simulink model "asm_blocks_lib"  (R2026b)
settings: Solver=VariableStepAuto
libraries: nesl_utility x45, asmlib_lib x25, fl_lib x3, ee_lib x3
(part 1 of 3)
settings Model: Creator=fsbb  LastModifiedBy=fsbb

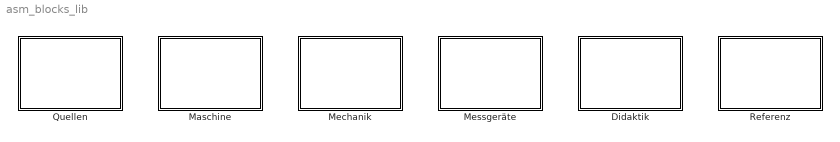
== system asm_blocks_lib ==
  Didaktik : Subsystem
      mask Display: disp('Didaktik');
  Maschine : Subsystem
      mask Display: disp('Maschine');
  Mechanik : Subsystem
      mask Display: disp('Mechanik');
  Messgeräte : Subsystem
      mask Display: disp('Messgeräte');
  Quellen : Subsystem
      mask Display: disp('Quellen');
  Referenz : Subsystem
      mask Display: disp('Referenz');

== system asm_blocks_lib/Didaktik ==
  Drehfeld-Anzeige : Subsystem  Tag=asmlib:field_display  mask(ASM-Bibliothek: Drehfeld-Anzeige){view_frame=rotorfest, image_orientation=wie Folien (U1 oben, Feld im Uhrzeigersinn), decomposition=on, change_vector=on, force_arrows=on, all_bars=on, slow_motion=0.05, N2=28, p=2, l=0.15, r=0.06, N1xi1=144, bar1_angle=-90}
      mask prompts: view_frame "Ansicht"; image_orientation "Orientierung"; decomposition "Feldzerlegung B⊥ / B∥ zeigen (Folie 16)"; change_vector "Änderungsvektor zeigen (Folie 17)"; force_arrows "Kraftpfeile zeigen (Folie 19)"; all_bars "alle Stäbe zeigen"; slow_motion "Zeitlupe (Simulationszeit je Sekunde Abspielzeit) [s]"; N2 "Anzahl Rotorstäbe N2 (2 = nur die Leiterschleife) [-]"; p "Polpaarzahl p [-]"; l "wirksame Stablänge l [m]"; r "Radius der Stabmitte r [m]"; N1xi1 "wirksame Windungszahl N1·ξ1 [-]"; bar1_angle "mechanische Lage von Stab 1 (0 = Achse Strang U, −90 = in der Folienansicht oben) [°]"
      mask help:
      | Rotorquerschnitt mit Drehfeld, Stabströmen und Kräften im Stil der Folien 16-30. Der Baustein
      | protokolliert ψh, i2′, ϑ in out.field_display_log (ein Baustein je Modell); nach der Simulation
      | startet der Knopf "Animation zeigen" die Animation (asmtools.field_animation). Einzelbilder
      | für Folien: asmexport.cross_section_series. Feldzerlegung und Änderungsvektor nur bei p = 1.
      |
      | Gleichungen:
      |   φ_el = ∠ψh,   B̂ = p·|ψh| / (2·N1ξ1·l·r),   B(γ,t) = B̂·cos(γ − φ_el)
      |   γ_k = p·ϑ + (k−1)·2π·p/N2,   î_Stab = 6·N1ξ1/N2·|i2′|,   ε2 = ∠i2′
      |   i_k = î_Stab·sin(γ_k − ε2) = î_Stab·sin(γ_k − φ_el + φ2),   φ2 = ∠ψh − ∠i2′
      |   B_k = B̂·cos(γ_k − φ_el),   F_k = i_k·l·B_k,   M_k = F_k·r
      |   Darstellung wie Folien: i_k,Folie = −i_k (positiv aus der Zeichenebene)
      |
      | Quelle: Hagl, R.: Elektrische Antriebstechnik. Hanser, München 2013; Densborn, Skript "DS-Asynchron-Motor" (DHBW Mannheim), Folien 16-30
      mask Help:
      | Rotorquerschnitt mit Drehfeld, Stabströmen und Kräften im Stil der Folien 16-30. Der Baustein
      | protokolliert ψh, i2′, ϑ in out.field_display_log (ein Baustein je Modell); nach der Simulation
      | startet der Knopf "Animation zeigen" die Animation (asmtools.field_animation). Einzelbilder
      | für Folien: asmexport.cross_section_series. Feldzerlegung und Änderungsvektor nur bei p = 1.
      | 
      | Gleichungen:
      |   φ_el = ∠ψh,   B̂ = p·|ψh| / (2·N1ξ1·l·r),   B(γ,t) = B̂·cos(γ − φ_el)
      |   γ_k = p·ϑ + (k−1)·2π·p/N2,   î_Stab = 6·N1ξ1/N2·|i2′|,   ε2 = ∠i2′
      |   i_k = î_Stab·sin(γ_k − ε2) = î_Stab·sin(γ_k − φ_el + φ2),   φ2 = ∠ψh − ∠i2′
      |   B_k = B̂·cos(γ_k − φ_el),   F_k = i_k·l·B_k,   M_k = F_k·r
      |   Darstellung wie Folien: i_k,Folie = −i_k (positiv aus der Zeichenebene)
      | 
      | Quelle: Hagl, R.: Elektrische Antriebstechnik. Hanser, München 2013; Densborn, Skript "DS-Asynchron-Motor" (DHBW Mannheim), Folien 16-30
      | 
      | Parameter und Wertebereiche:
      |   view_frame     Auswahl: rotorfest | statorfest
      |   image_orientation Auswahl: wie Folien (U1 oben, Feld im Uhrzeigersinn) | mathematisch positiv
      |   decomposition  ein/aus
      |   change_vector  ein/aus
      |   force_arrows   ein/aus
      |   all_bars       ein/aus
      |   slow_motion    > 0  [s]
      |   N2             ganzzahlig, ≥ 2  [-]
      |   p              ganzzahlig, ≥ 1, ≤ 12  [-]
      |   l              > 0  [m]
      |   r              > 0  [m]
      |   N1xi1          > 0  [-]
      |   bar1_angle     ≥ -360, ≤ 360  [°]
      | 
      | Alle Standardwerte sind Beispielwerte (parameter/asm_standard.m), keine Datenblattwerte.
      | Spezifikation: doku/SPEC.md
      mask TypeOptions view_frame: rotorfest | statorfest
      mask TypeOptions image_orientation: wie Folien (U1 oben, Feld im Uhrzeigersinn) | mathematisch positiv
      mask DialogControl evaluation_button Prompt: Animation zeigen
      mask DialogControl evaluation_button Callback: asmtools.field_animation(gcb);
      mask Display:
      | plot([0.1 0.9 0.9 0.1 0.1], [0.15 0.15 0.85 0.85 0.15]);
      | text(0.5, 0.5, 'Anzeige', 'horizontalAlignment', 'center', 'verticalAlignment', 'middle', 'texmode', 'on');
      | port_label('input', 1, '\psi_h', 'texmode', 'on');
      | port_label('input', 2, 'i2b', 'texmode', 'on');
      | port_label('input', 3, '\vartheta_{mech}', 'texmode', 'on');
  Ideales Drehfeld : Subsystem  Tag=asmlib:ideal_field  mask(ASM-Bibliothek: Ideales Drehfeld){Bhat=0.8, f1=50, p=2, s=1, l=0.15, r=0.06, N1xi1=144, N2=28, R2_S=0.000318664, L2s_S=5.0717e-06, phi2_mode=aus Rotorimpedanz (φ2 = 90° + φZ), phi2_fix=90}
      mask prompts: Bhat "Amplitude der Luftspaltflussdichte B̂ [T]"; f1 "Statorfrequenz f1 [Hz]"; p "Polpaarzahl p [-]"; s "Schlupf s [-]"; l "wirksame Stablänge l [m]"; r "Radius der Stabmitte r [m]"; N1xi1 "wirksame Windungszahl N1·ξ1 [-]"; N2 "Anzahl Rotorstäbe N2 (2 = nur die Leiterschleife) [-]"; R2_S "Widerstand einer Leiterschleife R2 [Ω]"; L2s_S "Streuinduktivität einer Leiterschleife L2σ [H]"; phi2_mode "Versatzwinkel φ2"; phi2_fix "fester Versatzwinkel φ2 [°]"
      mask help:
      | Kinematische Quelle wie Teil A des Prototyps: Drehfeld mit konstanter Amplitude, Rotor mit festem Schlupf.
      | Liefert dieselben Signale wie der Motor (ψh, i2′, ϑ), damit Rotorstab-Sonde und Drehfeld-Anzeige
      | ohne Motor betrieben werden können (Folien 16-30: s = 1, φ2 = 90°).
      |
      | Gleichungen:
      |   θ2 = ∫ s·ω1 dt,  U20 = 2·B̂·l·ω1·r/p,  î2 = s·U20/√(R2² + (s·ω1·L2σ)²)
      |   φZ = arctan(s·ω1·L2σ/R2),  φ2 = 90° + φZ  oder  φ2 = φ2,fix
      |
      | Quelle: Hagl, R.: Elektrische Antriebstechnik. Hanser, München 2013; Densborn, Skript "DS-Asynchron-Motor" (DHBW Mannheim), Folien 14-30
      mask Help:
      | Kinematische Quelle wie Teil A des Prototyps: Drehfeld mit konstanter Amplitude, Rotor mit festem Schlupf.
      | Liefert dieselben Signale wie der Motor (ψh, i2′, ϑ), damit Rotorstab-Sonde und Drehfeld-Anzeige
      | ohne Motor betrieben werden können (Folien 16-30: s = 1, φ2 = 90°).
      | 
      | Gleichungen:
      |   θ2 = ∫ s·ω1 dt,  U20 = 2·B̂·l·ω1·r/p,  î2 = s·U20/√(R2² + (s·ω1·L2σ)²)
      |   φZ = arctan(s·ω1·L2σ/R2),  φ2 = 90° + φZ  oder  φ2 = φ2,fix
      | 
      | Quelle: Hagl, R.: Elektrische Antriebstechnik. Hanser, München 2013; Densborn, Skript "DS-Asynchron-Motor" (DHBW Mannheim), Folien 14-30
      | 
      | Parameter und Wertebereiche:
      |   Bhat           > 0, ≤ 2.5  [T]
      |   f1             > 0, ≤ 1000  [Hz]
      |   p              ganzzahlig, ≥ 1, ≤ 12  [-]
      |   s              ≥ -1, ≤ 2  [-]
      |   l              > 0  [m]
      |   r              > 0  [m]
      |   N1xi1          > 0  [-]
      |   N2             ganzzahlig, ≥ 2  [-]
      |   R2_S           > 0  [Ω]
      |   L2s_S          > 0  [H]
      |   phi2_mode      Auswahl: aus Rotorimpedanz (φ2 = 90° + φZ) | fest
      |   phi2_fix       ≥ 0, ≤ 180  [°]
      | 
      | Alle Standardwerte sind Beispielwerte (parameter/asm_standard.m), keine Datenblattwerte.
      | Spezifikation: doku/SPEC.md
      mask TypeOptions phi2_mode: aus Rotorimpedanz (φ2 = 90° + φZ) | fest
      mask Display:
      | plot([0.1 0.9 0.9 0.1 0.1], [0.15 0.15 0.85 0.85 0.15]);
      | text(0.5, 0.5, 'Drehfeld', 'horizontalAlignment', 'center', 'verticalAlignment', 'middle', 'texmode', 'on');
      | port_label('output', 1, '\psi_h', 'texmode', 'on');
      | port_label('output', 2, 'i2b', 'texmode', 'on');
      | port_label('output', 3, '\vartheta_{mech}', 'texmode', 'on');
      | port_label('output', 4, '\phi_{el}', 'texmode', 'on');
      | port_label('output', 5, '\phi2', 'texmode', 'on');
  Kennlinienschreiber : Subsystem  Tag=asmlib:torque_speed_recorder  mask(ASM-Bibliothek: Kennlinienschreiber){show_kloss=on, show_ec=off, MK=71.55, sK=0.2, ns=1500}
      mask prompts: show_kloss "Kloss-Kennlinie einzeichnen"; show_ec "stationäre ESB-Kennlinie einzeichnen"; MK "Kippmoment MK [N·m]"; sK "Kippschlupf sK [-]"; ns "Synchrondrehzahl ns [1/min]"
      mask help:
      | Protokolliert n, M und M_L in out.torque_speed_log (ein Baustein je Modell). Der Knopf "Kennlinie
      | zeichnen" zeigt nach der Simulation das M(n)-Diagramm mit stationären Kennlinien und
      | Arbeitspunkt (asmtools.torque_speed_plot).
      |
      | Gleichungen:
      |   M = 2·MK·s·sK / (s² + sK²),   s = (ns − n)/ns
      |
      | Quelle: Hagl, R.: Elektrische Antriebstechnik. Hanser, München 2013; Densborn, Skript "DS-Asynchron-Motor" (DHBW Mannheim), Folien 47-56
      mask Help:
      | Protokolliert n, M und M_L in out.torque_speed_log (ein Baustein je Modell). Der Knopf "Kennlinie
      | zeichnen" zeigt nach der Simulation das M(n)-Diagramm mit stationären Kennlinien und
      | Arbeitspunkt (asmtools.torque_speed_plot).
      | 
      | Gleichungen:
      |   M = 2·MK·s·sK / (s² + sK²),   s = (ns − n)/ns
      | 
      | Quelle: Hagl, R.: Elektrische Antriebstechnik. Hanser, München 2013; Densborn, Skript "DS-Asynchron-Motor" (DHBW Mannheim), Folien 47-56
      | 
      | Parameter und Wertebereiche:
      |   show_kloss     ein/aus
      |   show_ec        ein/aus
      |   MK             > 0  [N·m]
      |   sK             > 0, ≤ 1  [-]
      |   ns             > 0  [1/min]
      | 
      | Alle Standardwerte sind Beispielwerte (parameter/asm_standard.m), keine Datenblattwerte.
      | Spezifikation: doku/SPEC.md
      mask DialogControl evaluation_button Prompt: Kennlinie zeichnen
      mask DialogControl evaluation_button Callback: asmtools.torque_speed_plot(gcb);
      mask Display:
      | plot([0.1 0.9 0.9 0.1 0.1], [0.15 0.15 0.85 0.85 0.15]);
      | text(0.5, 0.5, 'M(n)', 'horizontalAlignment', 'center', 'verticalAlignment', 'middle', 'texmode', 'on');
      | port_label('input', 1, 'n', 'texmode', 'on');
      | port_label('input', 2, 'M', 'texmode', 'on');
      | port_label('input', 3, 'M_L', 'texmode', 'on');
  Rotorstab-Sonde : Subsystem  Tag=asmlib:rotor_bar_probe  mask(ASM-Bibliothek: Rotorstab-Sonde){k1=1, k2=8, N2=28, p=2, l=0.15, r=0.06, N1xi1=144, bar1_angle=-90, convention=wie Folien (Strom aus der Zeichenebene positiv)}
      mask prompts: k1 "Nummer Stab 1 [-]"; k2 "Nummer Stab 2 (Standard: eine Polteilung weiter) [-]"; N2 "Anzahl Rotorstäbe N2 (2 = nur die Leiterschleife) [-]"; p "Polpaarzahl p [-]"; l "wirksame Stablänge l [m]"; r "Radius der Stabmitte r [m]"; N1xi1 "wirksame Windungszahl N1·ξ1 [-]"; bar1_angle "mechanische Lage von Stab 1 (0 = Achse Strang U, −90 = in der Folienansicht oben) [°]"; convention "Zählrichtung des Stabstroms"
      mask help:
      | Berechnet Flussdichte, Strom, Kraft und Moment an zwei Rotorstäben (Leiterschleife wie Folie 16)
      | aus den Modellgrößen ψh, i2′ und ϑ. M_sum ist die Summe über alle N2 Stäbe (Kontrolle: M_sum = M).
      |
      | Gleichungen:
      |   φ_el = ∠ψh,   B̂ = p·|ψh| / (2·N1ξ1·l·r),   B(γ,t) = B̂·cos(γ − φ_el)
      |   γ_k = p·ϑ + (k−1)·2π·p/N2,   î_Stab = 6·N1ξ1/N2·|i2′|,   ε2 = ∠i2′
      |   i_k = î_Stab·sin(γ_k − ε2) = î_Stab·sin(γ_k − φ_el + φ2),   φ2 = ∠ψh − ∠i2′
      |   B_k = B̂·cos(γ_k − φ_el),   F_k = i_k·l·B_k,   M_k = F_k·r
      |   Darstellung wie Folien: i_k,Folie = −i_k (positiv aus der Zeichenebene)
      |   B⊥ = B̂·sin(γ_1 − φ_el) (Folienzählung: −B̂·sin(γ_1 − φ_el)),  Σ M_k = 3/2·p·|ψh|·|i2′|·sin φ2 = M
      |
      | Quelle: Hagl, R.: Elektrische Antriebstechnik. Hanser, München 2013; Densborn, Skript "DS-Asynchron-Motor" (DHBW Mannheim), Folien 14-30
      mask Help:
      | Berechnet Flussdichte, Strom, Kraft und Moment an zwei Rotorstäben (Leiterschleife wie Folie 16)
      | aus den Modellgrößen ψh, i2′ und ϑ. M_sum ist die Summe über alle N2 Stäbe (Kontrolle: M_sum = M).
      | 
      | Gleichungen:
      |   φ_el = ∠ψh,   B̂ = p·|ψh| / (2·N1ξ1·l·r),   B(γ,t) = B̂·cos(γ − φ_el)
      |   γ_k = p·ϑ + (k−1)·2π·p/N2,   î_Stab = 6·N1ξ1/N2·|i2′|,   ε2 = ∠i2′
      |   i_k = î_Stab·sin(γ_k − ε2) = î_Stab·sin(γ_k − φ_el + φ2),   φ2 = ∠ψh − ∠i2′
      |   B_k = B̂·cos(γ_k − φ_el),   F_k = i_k·l·B_k,   M_k = F_k·r
      |   Darstellung wie Folien: i_k,Folie = −i_k (positiv aus der Zeichenebene)
      |   B⊥ = B̂·sin(γ_1 − φ_el) (Folienzählung: −B̂·sin(γ_1 − φ_el)),  Σ M_k = 3/2·p·|ψh|·|i2′|·sin φ2 = M
      | 
      | Quelle: Hagl, R.: Elektrische Antriebstechnik. Hanser, München 2013; Densborn, Skript "DS-Asynchron-Motor" (DHBW Mannheim), Folien 14-30
      | 
      | Parameter und Wertebereiche:
      |   k1             ganzzahlig, ≥ 1  [-]
      |   k2             ganzzahlig, ≥ 1  [-]
      |   N2             ganzzahlig, ≥ 2  [-]
      |   p              ganzzahlig, ≥ 1, ≤ 12  [-]
      |   l              > 0  [m]
      |   r              > 0  [m]
      |   N1xi1          > 0  [-]
      |   bar1_angle     ≥ -360, ≤ 360  [°]
      |   convention     Auswahl: wie Folien (Strom aus der Zeichenebene positiv) | rechtshändig (konv_phi2 = +1)
      | 
      | Alle Standardwerte sind Beispielwerte (parameter/asm_standard.m), keine Datenblattwerte.
      | Spezifikation: doku/SPEC.md
      mask TypeOptions convention: wie Folien (Strom aus der Zeichenebene positiv) | rechtshändig (konv_phi2 = +1)
      mask Display:
      | plot([0.1 0.9 0.9 0.1 0.1], [0.15 0.15 0.85 0.85 0.15]);
      | text(0.5, 0.5, 'Stab', 'horizontalAlignment', 'center', 'verticalAlignment', 'middle', 'texmode', 'on');
      | port_label('input', 1, '\psi_h', 'texmode', 'on');
      | port_label('input', 2, 'i2b', 'texmode', 'on');
      | port_label('input', 3, '\vartheta_{mech}', 'texmode', 'on');
      | port_label('output', 1, 'B_k', 'texmode', 'on');
      | port_label('output', 2, 'i_k', 'texmode', 'on');
      | port_label('output', 3, 'F_k', 'texmode', 'on');
      | port_label('output', 4, 'M_k', 'texmode', 'on');
      | port_label('output', 5, 'M_S', 'texmode', 'on');
      | port_label('output', 6, 'B_\perp', 'texmode', 'on');
      | port_label('output', 7, 'dB_\perp', 'texmode', 'on');
      | port_label('output', 8, 'sgn_i', 'texmode', 'on');
      | port_label('output', 9, '\phi2', 'texmode', 'on');
      | port_label('output', 10, 'M_{sum}', 'texmode', 'on');
  Spulenfelder : Subsystem  Tag=asmlib:coil_fields  mask(ASM-Bibliothek: Spulenfelder){Lh=0.25, N1xi1=144, p=2, l=0.15, r=0.06}
      mask prompts: Lh "Hauptinduktivität Lh [H]"; N1xi1 "wirksame Windungszahl N1·ξ1 [-]"; p "Polpaarzahl p [-]"; l "wirksame Stablänge l [m]"; r "Radius der Stabmitte r [m]"
      mask help:
      | Felder der Einzelspulen U, V, W und ihre Überlagerung zum Drehfeld (wie Hagl Bild 6.13).
      |
      | Gleichungen:
      |   B_U(γ,t) = B̂_Str(t)·sin γ,  B_V, B_W um 2π/3 bzw. 4π/3 versetzt
      |   B = B_U + B_V + B_W = 1,5·B̂_Str,max·cos(γ − φ_el)
      |
      | Quelle: Hagl, R.: Elektrische Antriebstechnik. Hanser, München 2013; Densborn, Skript "Drehstrom & Drehfeld" (DHBW Mannheim), Folien 55-62
      mask Help:
      | Felder der Einzelspulen U, V, W und ihre Überlagerung zum Drehfeld (wie Hagl Bild 6.13).
      | 
      | Gleichungen:
      |   B_U(γ,t) = B̂_Str(t)·sin γ,  B_V, B_W um 2π/3 bzw. 4π/3 versetzt
      |   B = B_U + B_V + B_W = 1,5·B̂_Str,max·cos(γ − φ_el)
      | 
      | Quelle: Hagl, R.: Elektrische Antriebstechnik. Hanser, München 2013; Densborn, Skript "Drehstrom & Drehfeld" (DHBW Mannheim), Folien 55-62
      | 
      | Parameter und Wertebereiche:
      |   Lh             > 0  [H]
      |   N1xi1          > 0  [-]
      |   p              ganzzahlig, ≥ 1, ≤ 12  [-]
      |   l              > 0  [m]
      |   r              > 0  [m]
      | 
      | Alle Standardwerte sind Beispielwerte (parameter/asm_standard.m), keine Datenblattwerte.
      | Spezifikation: doku/SPEC.md
      mask Display:
      | plot([0.1 0.9 0.9 0.1 0.1], [0.15 0.15 0.85 0.85 0.15]);
      | text(0.5, 0.5, 'B_U B_V B_W', 'horizontalAlignment', 'center', 'verticalAlignment', 'middle', 'texmode', 'on');
      | port_label('input', 1, 'i_{abc}', 'texmode', 'on');
      | port_label('output', 1, 'B_{UVW}', 'texmode', 'on');
      | port_label('output', 2, 'Bhat', 'texmode', 'on');
      | port_label('output', 3, '\phi_{el}', 'texmode', 'on');

== system asm_blocks_lib/Maschine ==
  ASM Standard : Subsystem  Tag=asmlib:asm_standard  mask(ASM-Bibliothek: ASM Standard){param_set=Standard, connection=Stern, U_N=400, f_N=50, p=2, R1=0.5, L1s=0.009902, Lh=0.25, R2b=1.225, L2sb=0.009902, J_M=0.012, k_R=0, n0=0, l=0.15, r=0.06, N2=28, Bhat_N=0.8}
      mask prompts: param_set "Parametersatz"; connection "Schaltung der Statorwicklung"; U_N "Bemessungsspannung U_N (Leiter, eff.) [V]"; f_N "Bemessungsfrequenz f_N [Hz]"; p "Polpaarzahl p [-]"; R1 "Statorwiderstand R1 [Ω]"; L1s "Statorstreuinduktivität L1σ [H]"; Lh "Hauptinduktivität Lh [H]"; R2b "Rotorwiderstand R2′ (statorbezogen) [Ω]"; L2sb "Rotorstreuinduktivität L2σ′ (statorbezogen) [H]"; J_M "Trägheitsmoment Motor J_M [kg·m²]"; k_R "Reibbeiwert k_R (viskos) [N·m·s/rad]"; n0 "Anfangsdrehzahl n0 [1/min]"; l "wirksame Stablänge l [m]"; r "Radius der Stabmitte r [m]"; N2 "Anzahl Rotorstäbe N2 [-]"; Bhat_N "Luftspaltflussdichte im Bemessungspunkt B̂_N [T]"
      mask help:
      | Drehstrom-Asynchronmotor mit Käfigläufer, dynamisches Raumzeigermodell.
      | Parametersatz "Standard": Beispielmotor 4 kW, 4-polig (keine Datenblattwerte). Erst bei
      | "Benutzerdefiniert" sind die Felder editierbar. Unter der Maske (Ctrl+U) liegt der zerlegte
      | Motor: Klemmbrett, Stator, Luftspalt-Drehfeld, Käfigläufer.
      | Ausgang Mess (Bus): i1, u1, psi_h, phi_el, Bhat, i_mu, i2b, M, n, Om, th_mech, theta2, s.
      | N1ξ1 wird aus B̂_N bestimmt: N1ξ1 = p·(U_N/√3·√2/ω_N)/(2·B̂_N·l·r).
      |
      | Gleichungen:
      | Raumzeigermodell, statorfest (Index 1 = Stator, 2 = Rotor, ′ = statorbezogen):
      |   u1 = R1·i1 + dψ1/dt
      |   0  = R2′·i2′ + dψ2′/dt − j·p·Ω·ψ2′
      |   ψ1 = L1σ·i1 + ψh,   ψ2′ = L2σ′·i2′ + ψh,   ψh = Lh·(i1 + i2′)
      |   M  = 3/2·p·Im{ψh*·i1},   J·dΩ/dt = M − M_L − k_R·Ω
      |   n = 60·Ω/(2π),   s = (ns − n)/ns,   ns = 60·f1/p
      |   φ_el = ∠ψh,   B̂ = p·|ψh| / (2·N1ξ1·l·r),   B(γ,t) = B̂·cos(γ − φ_el)
      |
      | Quelle: Hagl, R.: Elektrische Antriebstechnik. Hanser, München 2013; Densborn, Skript "DS-Asynchron-Motor" (DHBW Mannheim), Folien 14-16
      mask init:
      | % parameter set "Standard": values from parameter/asm_standard.m
      | if param_set == 1
      |     S = asm_standard();
      |     U_N = S.U_N; f_N = S.f_N; p = S.p; R1 = S.R1; L1s = S.L1s; Lh = S.Lh; R2b = S.R2b; L2sb = S.L2sb; J_M = S.J_M; k_R = S.k_R; l = S.l; r = S.r; N2 = S.N2; Bhat_N = S.Bhat_N;
      | end
      | % effective number of turns from the air-gap flux density at the rated point
      | N1xi1 = p*(U_N/sqrt(3)*sqrt(2)/(2*pi*f_N))/(2*Bhat_N*l*r);
      mask Help:
      | Drehstrom-Asynchronmotor mit Käfigläufer, dynamisches Raumzeigermodell.
      | Parametersatz "Standard": Beispielmotor 4 kW, 4-polig (keine Datenblattwerte). Erst bei
      | "Benutzerdefiniert" sind die Felder editierbar. Unter der Maske (Ctrl+U) liegt der zerlegte
      | Motor: Klemmbrett, Stator, Luftspalt-Drehfeld, Käfigläufer.
      | Ausgang Mess (Bus): i1, u1, psi_h, phi_el, Bhat, i_mu, i2b, M, n, Om, th_mech, theta2, s.
      | N1ξ1 wird aus B̂_N bestimmt: N1ξ1 = p·(U_N/√3·√2/ω_N)/(2·B̂_N·l·r).
      | 
      | Gleichungen:
      | Raumzeigermodell, statorfest (Index 1 = Stator, 2 = Rotor, ′ = statorbezogen):
      |   u1 = R1·i1 + dψ1/dt
      |   0  = R2′·i2′ + dψ2′/dt − j·p·Ω·ψ2′
      |   ψ1 = L1σ·i1 + ψh,   ψ2′ = L2σ′·i2′ + ψh,   ψh = Lh·(i1 + i2′)
      |   M  = 3/2·p·Im{ψh*·i1},   J·dΩ/dt = M − M_L − k_R·Ω
      |   n = 60·Ω/(2π),   s = (ns − n)/ns,   ns = 60·f1/p
      |   φ_el = ∠ψh,   B̂ = p·|ψh| / (2·N1ξ1·l·r),   B(γ,t) = B̂·cos(γ − φ_el)
      | 
      | Quelle: Hagl, R.: Elektrische Antriebstechnik. Hanser, München 2013; Densborn, Skript "DS-Asynchron-Motor" (DHBW Mannheim), Folien 14-16
      | 
      | Parameter und Wertebereiche:
      |   param_set      Auswahl: Standard | Benutzerdefiniert
      |   connection     Auswahl: Stern | Dreieck
      |   U_N            > 0, ≤ 1e4  [V]
      |   f_N            > 0, ≤ 1000  [Hz]
      |   p              ganzzahlig, ≥ 1, ≤ 12  [-]
      |   R1             > 0  [Ω]
      |   L1s            > 0  [H]
      |   Lh             > 0  [H]
      |   R2b            > 0  [Ω]
      |   L2sb           > 0  [H]
      |   J_M            > 0  [kg·m²]
      |   k_R            ≥ 0  [N·m·s/rad]
      |   n0             endlich  [1/min]
      |   l              > 0  [m]
      |   r              > 0  [m]
      |   N2             ganzzahlig, ≥ 3  [-]
      |   Bhat_N         > 0, ≤ 2.5  [T]
      | 
      | Alle Standardwerte sind Beispielwerte (parameter/asm_standard.m), keine Datenblattwerte.
      | Spezifikation: doku/SPEC.md
      mask TypeOptions param_set: Standard | Benutzerdefiniert
      mask Callback param_set: asmtools.param_set_callback(gcb);
      mask TypeOptions connection: Stern | Dreieck
      mask Display:
      | plot(0.5+0.36*cos(0:0.05:6.3), 0.5+0.36*sin(0:0.05:6.3));
      | plot(0.5+0.26*cos(0:0.05:6.3), 0.5+0.26*sin(0:0.05:6.3));
      | text(0.5, 0.5, 'M 3~', 'horizontalAlignment', 'center', 'verticalAlignment', 'middle', 'texmode', 'on');
      | port_label('LConn', 1, 'a', 'texmode', 'on');
      | port_label('LConn', 2, 'b', 'texmode', 'on');
      | port_label('LConn', 3, 'c', 'texmode', 'on');
      | port_label('RConn', 1, 'R', 'texmode', 'on');
      | port_label('RConn', 2, 'C', 'texmode', 'on');
      | port_label('output', 1, 'Mess', 'texmode', 'on');
  Klemmbrett : Subsystem  Tag=asmlib:terminal_box  mask(ASM-Bibliothek: Klemmbrett){connection=Stern}
      mask prompts: connection "Schaltung der Statorwicklung"
      mask help:
      | Klemmenkasten: verbindet die Netzleiter a, b, c mit den Wicklungsenden in Stern- oder Dreieckschaltung.
      |
      | Gleichungen:
      |   Stern:   a-U1, b-V1, c-W1, U2 = V2 = W2 (Sternpunkt)
      |   Dreieck: a-U1-W2, b-V1-U2, c-W1-V2
      |
      | Quelle: Hagl, R.: Elektrische Antriebstechnik. Hanser, München 2013; Densborn, Skript "Drehstrom & Drehfeld" (DHBW Mannheim), Folien 23-26
      mask Help:
      | Klemmenkasten: verbindet die Netzleiter a, b, c mit den Wicklungsenden in Stern- oder Dreieckschaltung.
      | 
      | Gleichungen:
      |   Stern:   a-U1, b-V1, c-W1, U2 = V2 = W2 (Sternpunkt)
      |   Dreieck: a-U1-W2, b-V1-U2, c-W1-V2
      | 
      | Quelle: Hagl, R.: Elektrische Antriebstechnik. Hanser, München 2013; Densborn, Skript "Drehstrom & Drehfeld" (DHBW Mannheim), Folien 23-26
      | 
      | Parameter und Wertebereiche:
      |   connection     Auswahl: Stern | Dreieck
      | 
      | Alle Standardwerte sind Beispielwerte (parameter/asm_standard.m), keine Datenblattwerte.
      | Spezifikation: doku/SPEC.md
      mask TypeOptions connection: Stern | Dreieck
      mask Display:
      | plot(0.5+0.36*cos(0:0.05:6.3), 0.5+0.36*sin(0:0.05:6.3));
      | plot(0.5+0.26*cos(0:0.05:6.3), 0.5+0.26*sin(0:0.05:6.3));
      | text(0.5, 0.5, 'Y / \Delta', 'horizontalAlignment', 'center', 'verticalAlignment', 'middle', 'texmode', 'on');
      | port_label('LConn', 1, 'a', 'texmode', 'on');
      | port_label('LConn', 2, 'b', 'texmode', 'on');
      | port_label('LConn', 3, 'c', 'texmode', 'on');
      | port_label('RConn', 1, 'U1', 'texmode', 'on');
      | port_label('RConn', 2, 'V1', 'texmode', 'on');
      | port_label('RConn', 3, 'W1', 'texmode', 'on');
      | port_label('RConn', 4, 'U2', 'texmode', 'on');
      | port_label('RConn', 5, 'V2', 'texmode', 'on');
      | port_label('RConn', 6, 'W2', 'texmode', 'on');
  Käfigläufer : Subsystem  Tag=asmlib:squirrel_cage  mask(ASM-Bibliothek: Käfigläufer){R2b=1.225, L2sb=0.009902, p=2, f_N=50, J_M=0.012, k_R=0, n0=0}
      mask prompts: R2b "Rotorwiderstand R2′ (statorbezogen) [Ω]"; L2sb "Rotorstreuinduktivität L2σ′ (statorbezogen) [H]"; p "Polpaarzahl p [-]"; f_N "Bemessungsfrequenz f_N [Hz]"; J_M "Trägheitsmoment Motor J_M [kg·m²]"; k_R "Reibbeiwert k_R (viskos) [N·m·s/rad]"; n0 "Anfangsdrehzahl n0 [1/min]"
      mask help:
      | Kurzgeschlossener Käfig (statorbezogene Rotorgrößen) mit Welle (R) und Gehäuse (C).
      |
      | Gleichungen:
      |   0 = R2′·i2′ + dψ2′/dt − j·p·Ω·ψ2′,  ψ2′ = L2σ′·i2′ + ψh
      |   M = −3/2·p·Im{ψ2′*·i2′},  J_M·dΩ/dt = M − M_Welle − k_R·Ω
      |   θ2 = φ_el − p·ϑ,  s = (ns − n)/ns
      |
      | Quelle: Hagl, R.: Elektrische Antriebstechnik. Hanser, München 2013
      mask Help:
      | Kurzgeschlossener Käfig (statorbezogene Rotorgrößen) mit Welle (R) und Gehäuse (C).
      | 
      | Gleichungen:
      |   0 = R2′·i2′ + dψ2′/dt − j·p·Ω·ψ2′,  ψ2′ = L2σ′·i2′ + ψh
      |   M = −3/2·p·Im{ψ2′*·i2′},  J_M·dΩ/dt = M − M_Welle − k_R·Ω
      |   θ2 = φ_el − p·ϑ,  s = (ns − n)/ns
      | 
      | Quelle: Hagl, R.: Elektrische Antriebstechnik. Hanser, München 2013
      | 
      | Parameter und Wertebereiche:
      |   R2b            > 0  [Ω]
      |   L2sb           > 0  [H]
      |   p              ganzzahlig, ≥ 1, ≤ 12  [-]
      |   f_N            > 0, ≤ 1000  [Hz]
      |   J_M            > 0  [kg·m²]
      |   k_R            ≥ 0  [N·m·s/rad]
      |   n0             endlich  [1/min]
      | 
      | Alle Standardwerte sind Beispielwerte (parameter/asm_standard.m), keine Datenblattwerte.
      | Spezifikation: doku/SPEC.md
      mask Display:
      | plot(0.5+0.36*cos(0:0.05:6.3), 0.5+0.36*sin(0:0.05:6.3));
      | plot(0.5+0.26*cos(0:0.05:6.3), 0.5+0.26*sin(0:0.05:6.3));
      | text(0.5, 0.5, 'Käfig', 'horizontalAlignment', 'center', 'verticalAlignment', 'middle', 'texmode', 'on');
      | port_label('LConn', 1, 'LS', 'texmode', 'on');
      | port_label('RConn', 1, 'R', 'texmode', 'on');
      | port_label('RConn', 2, 'C', 'texmode', 'on');
      | port_label('output', 1, 'i2b', 'texmode', 'on');
      | port_label('output', 2, 'M', 'texmode', 'on');
      | port_label('output', 3, 'Om', 'texmode', 'on');
      | port_label('output', 4, '\vartheta_{mech}', 'texmode', 'on');
      | port_label('output', 5, '\theta_2', 'texmode', 'on');
      | port_label('output', 6, 's', 'texmode', 'on');
  Luftspalt-Drehfeld : Subsystem  Tag=asmlib:airgap_field  mask(ASM-Bibliothek: Luftspalt-Drehfeld){Lh=0.25, p=2, N1xi1=144, l=0.15, r=0.06}
      mask prompts: Lh "Hauptinduktivität Lh [H]"; p "Polpaarzahl p [-]"; N1xi1 "wirksame Windungszahl N1·ξ1 [-]"; l "wirksame Stablänge l [m]"; r "Radius der Stabmitte r [m]"
      mask help:
      | Luftspalt mit Hauptinduktivität. Liefert das Drehfeld (Lage φ_el und Amplitude B̂ der Luftspaltflussdichte).
      |
      | Gleichungen:
      |   ψh = Lh·iμ,  iμ = i1 + i2′  (Durchflutungsbilanz am Port LS)
      |   φ_el = ∠ψh,   B̂ = p·|ψh| / (2·N1ξ1·l·r),   B(γ,t) = B̂·cos(γ − φ_el)
      |
      | Quelle: Hagl, R.: Elektrische Antriebstechnik. Hanser, München 2013; Densborn, Skript "Drehstrom & Drehfeld" (DHBW Mannheim), Folien 59-62; Hagl, R.: Elektrische Antriebstechnik. Hanser, München 2013; Densborn, Skript "DS-Asynchron-Motor" (DHBW Mannheim), Folie 14
      mask Help:
      | Luftspalt mit Hauptinduktivität. Liefert das Drehfeld (Lage φ_el und Amplitude B̂ der Luftspaltflussdichte).
      | 
      | Gleichungen:
      |   ψh = Lh·iμ,  iμ = i1 + i2′  (Durchflutungsbilanz am Port LS)
      |   φ_el = ∠ψh,   B̂ = p·|ψh| / (2·N1ξ1·l·r),   B(γ,t) = B̂·cos(γ − φ_el)
      | 
      | Quelle: Hagl, R.: Elektrische Antriebstechnik. Hanser, München 2013; Densborn, Skript "Drehstrom & Drehfeld" (DHBW Mannheim), Folien 59-62; Hagl, R.: Elektrische Antriebstechnik. Hanser, München 2013; Densborn, Skript "DS-Asynchron-Motor" (DHBW Mannheim), Folie 14
      | 
      | Parameter und Wertebereiche:
      |   Lh             > 0  [H]
      |   p              ganzzahlig, ≥ 1, ≤ 12  [-]
      |   N1xi1          > 0  [-]
      |   l              > 0  [m]
      |   r              > 0  [m]
      | 
      | Alle Standardwerte sind Beispielwerte (parameter/asm_standard.m), keine Datenblattwerte.
      | Spezifikation: doku/SPEC.md
      mask Display:
      | plot(0.5+0.36*cos(0:0.05:6.3), 0.5+0.36*sin(0:0.05:6.3));
      | plot(0.5+0.26*cos(0:0.05:6.3), 0.5+0.26*sin(0:0.05:6.3));
      | text(0.5, 0.5, 'B(\gamma,t)', 'horizontalAlignment', 'center', 'verticalAlignment', 'middle', 'texmode', 'on');
      | port_label('LConn', 1, 'LS', 'texmode', 'on');
      | port_label('output', 1, '\psi_h', 'texmode', 'on');
      | port_label('output', 2, '\phi_{el}', 'texmode', 'on');
      | port_label('output', 3, 'Bhat', 'texmode', 'on');
      | port_label('output', 4, 'i_\mu', 'texmode', 'on');
  Stator : Subsystem  Tag=asmlib:stator  mask(ASM-Bibliothek: Stator){R1=0.5, L1s=0.009902}
      mask prompts: R1 "Statorwiderstand R1 [Ω]"; L1s "Statorstreuinduktivität L1σ [H]"
      mask help:
      | Statorwicklung (drei Stränge U1-U2, V1-V2, W1-W2) mit Widerstand und Streuinduktivität. Der Port LS koppelt an den Luftspalt.
      |
      | Gleichungen:
      |   u1 = R1·i1 + L1σ·di1/dt + dψh/dt   (Raumzeiger, αβ)
      |   i1 = 2/3·(i_U + a·i_V + a²·i_W),  a = e^(j2π/3)
      |
      | Quelle: Hagl, R.: Elektrische Antriebstechnik. Hanser, München 2013
      mask Help:
      | Statorwicklung (drei Stränge U1-U2, V1-V2, W1-W2) mit Widerstand und Streuinduktivität. Der Port LS koppelt an den Luftspalt.
      | 
      | Gleichungen:
      |   u1 = R1·i1 + L1σ·di1/dt + dψh/dt   (Raumzeiger, αβ)
      |   i1 = 2/3·(i_U + a·i_V + a²·i_W),  a = e^(j2π/3)
      | 
      | Quelle: Hagl, R.: Elektrische Antriebstechnik. Hanser, München 2013
      | 
      | Parameter und Wertebereiche:
      |   R1             > 0  [Ω]
      |   L1s            > 0  [H]
      | 
      | Alle Standardwerte sind Beispielwerte (parameter/asm_standard.m), keine Datenblattwerte.
      | Spezifikation: doku/SPEC.md
      mask Display:
      | plot(0.5+0.36*cos(0:0.05:6.3), 0.5+0.36*sin(0:0.05:6.3));
      | plot(0.5+0.26*cos(0:0.05:6.3), 0.5+0.26*sin(0:0.05:6.3));
      | text(0.5, 0.5, 'Stator', 'horizontalAlignment', 'center', 'verticalAlignment', 'middle', 'texmode', 'on');
      | port_label('LConn', 1, 'U1', 'texmode', 'on');
      | port_label('LConn', 2, 'V1', 'texmode', 'on');
      | port_label('LConn', 3, 'W1', 'texmode', 'on');
      | port_label('LConn', 4, 'U2', 'texmode', 'on');
      | port_label('LConn', 5, 'V2', 'texmode', 'on');
      | port_label('LConn', 6, 'W2', 'texmode', 'on');
      | port_label('RConn', 1, 'LS', 'texmode', 'on');
      | port_label('output', 1, 'i1', 'texmode', 'on');
      | port_label('output', 2, 'u1', 'texmode', 'on');

== system asm_blocks_lib/Mechanik ==
  Last Kennlinie : Subsystem  Tag=asmlib:load_table  mask(ASM-Bibliothek: Last Kennlinie){n_tab=[0 1500], M_tab=[0 26.5]}
      mask prompts: n_tab "Stützstellen Drehzahl n [1/min]"; M_tab "Stützstellen Lastmoment M_L [N·m]"
      mask help:
      | Lastkennlinie aus einer Tabelle (lineare Interpolation), wirkt stets gegen die Drehrichtung.
      |
      | Gleichungen:
      |   M_L = interp1(n_tab, M_tab, |n|)·sign(n)
      |
      | Quelle: Hagl, R.: Elektrische Antriebstechnik. Hanser, München 2013; Densborn, Skript "DS-Asynchron-Motor" (DHBW Mannheim), Folien 47-56
      mask Help:
      | Lastkennlinie aus einer Tabelle (lineare Interpolation), wirkt stets gegen die Drehrichtung.
      | 
      | Gleichungen:
      |   M_L = interp1(n_tab, M_tab, |n|)·sign(n)
      | 
      | Quelle: Hagl, R.: Elektrische Antriebstechnik. Hanser, München 2013; Densborn, Skript "DS-Asynchron-Motor" (DHBW Mannheim), Folien 47-56
      | 
      | Parameter und Wertebereiche:
      |   n_tab          Vektor, ≥ 0  [1/min]
      |   M_tab          Vektor, ≥ 0  [N·m]
      | 
      | Alle Standardwerte sind Beispielwerte (parameter/asm_standard.m), keine Datenblattwerte.
      | Spezifikation: doku/SPEC.md
      mask Display:
      | plot([0.05 0.95], [0.5 0.5]);
      | text(0.5, 0.5, 'M_L', 'horizontalAlignment', 'center', 'verticalAlignment', 'middle', 'texmode', 'on');
      | port_label('LConn', 1, 'R', 'texmode', 'on');
      | port_label('RConn', 1, 'C', 'texmode', 'on');
  Last Lüfter : Subsystem  Tag=asmlib:load_fan  mask(ASM-Bibliothek: Last Lüfter){M_B=26.5, n_B=1440}
      mask prompts: M_B "Bezugsmoment M_B [N·m]"; n_B "Bezugsdrehzahl n_B [1/min]"
      mask help:
      | Quadratische Lastkennlinie (Lüfter, Pumpe), wirkt stets gegen die Drehrichtung.
      |
      | Gleichungen:
      |   M_L = M_B·(n/n_B)·|n/n_B|
      |
      | Quelle: Hagl, R.: Elektrische Antriebstechnik. Hanser, München 2013; Densborn, Skript "DS-Asynchron-Motor" (DHBW Mannheim), Folien 47-56
      mask Help:
      | Quadratische Lastkennlinie (Lüfter, Pumpe), wirkt stets gegen die Drehrichtung.
      | 
      | Gleichungen:
      |   M_L = M_B·(n/n_B)·|n/n_B|
      | 
      | Quelle: Hagl, R.: Elektrische Antriebstechnik. Hanser, München 2013; Densborn, Skript "DS-Asynchron-Motor" (DHBW Mannheim), Folien 47-56
      | 
      | Parameter und Wertebereiche:
      |   M_B            ≥ 0  [N·m]
      |   n_B            > 0  [1/min]
      | 
      | Alle Standardwerte sind Beispielwerte (parameter/asm_standard.m), keine Datenblattwerte.
      | Spezifikation: doku/SPEC.md
      mask Display:
      | plot([0.05 0.95], [0.5 0.5]);
      | text(0.5, 0.5, 'M_L', 'horizontalAlignment', 'center', 'verticalAlignment', 'middle', 'texmode', 'on');
      | port_label('LConn', 1, 'R', 'texmode', 'on');
      | port_label('RConn', 1, 'C', 'texmode', 'on');
  Last konstant : Subsystem  Tag=asmlib:load_constant  mask(ASM-Bibliothek: Last konstant){M_L0=13.25}
      mask prompts: M_L0 "Lastmoment M_L0 [N·m]"
      mask help:
      | Konstantes Lastmoment, wirkt stets gegen die Drehrichtung (Hubwerk-/Förderband-Kennlinie).
      |
      | Gleichungen:
      |   M_L = M_L0·sign(Ω)  (bei Ω ≈ 0 geglättet)
      |
      | Quelle: Hagl, R.: Elektrische Antriebstechnik. Hanser, München 2013; Densborn, Skript "DS-Asynchron-Motor" (DHBW Mannheim), Folien 47-56
      mask Help:
      | Konstantes Lastmoment, wirkt stets gegen die Drehrichtung (Hubwerk-/Förderband-Kennlinie).
      | 
      | Gleichungen:
      |   M_L = M_L0·sign(Ω)  (bei Ω ≈ 0 geglättet)
      | 
      | Quelle: Hagl, R.: Elektrische Antriebstechnik. Hanser, München 2013; Densborn, Skript "DS-Asynchron-Motor" (DHBW Mannheim), Folien 47-56
      | 
      | Parameter und Wertebereiche:
      |   M_L0           ≥ 0  [N·m]
      | 
      | Alle Standardwerte sind Beispielwerte (parameter/asm_standard.m), keine Datenblattwerte.
      | Spezifikation: doku/SPEC.md
      mask Display:
      | plot([0.05 0.95], [0.5 0.5]);
      | text(0.5, 0.5, 'M_L', 'horizontalAlignment', 'center', 'verticalAlignment', 'middle', 'texmode', 'on');
      | port_label('LConn', 1, 'R', 'texmode', 'on');
      | port_label('RConn', 1, 'C', 'texmode', 'on');
  Laststoß : Subsystem  Tag=asmlib:load_step  mask(ASM-Bibliothek: Laststoß){t_step=1, dM_L=7.95}
      mask prompts: t_step "Zeitpunkt des Laststoßes t_stoß [s]"; dM_L "Höhe des Laststoßes ΔM_L [N·m]"
      mask help:
      | Sprungförmige Laständerung, wirkt gegen die Drehrichtung.
      |
      | Gleichungen:
      |   M_L = ΔM_L·σ(t − t_stoß)·sign(Ω)
      |
      | Quelle: Hagl, R.: Elektrische Antriebstechnik. Hanser, München 2013; Densborn, Skript "DS-Asynchron-Motor" (DHBW Mannheim), Folien 53-54
      mask Help:
      | Sprungförmige Laständerung, wirkt gegen die Drehrichtung.
      | 
      | Gleichungen:
      |   M_L = ΔM_L·σ(t − t_stoß)·sign(Ω)
      | 
      | Quelle: Hagl, R.: Elektrische Antriebstechnik. Hanser, München 2013; Densborn, Skript "DS-Asynchron-Motor" (DHBW Mannheim), Folien 53-54
      | 
      | Parameter und Wertebereiche:
      |   t_step         ≥ 0  [s]
      |   dM_L           endlich  [N·m]
      | 
      | Alle Standardwerte sind Beispielwerte (parameter/asm_standard.m), keine Datenblattwerte.
      | Spezifikation: doku/SPEC.md
      mask Display:
      | plot([0.05 0.95], [0.5 0.5]);
      | text(0.5, 0.5, '\DeltaM_L', 'horizontalAlignment', 'center', 'verticalAlignment', 'middle', 'texmode', 'on');
      | port_label('LConn', 1, 'R', 'texmode', 'on');
      | port_label('RConn', 1, 'C', 'texmode', 'on');
  Mechanischer Bezug : Subsystem  Tag=asmlib:mech_reference  mask(ASM-Bibliothek: Mechanischer Bezug){}
      mask help:
      | Ruhendes Bezugssystem (Fundament, Gehäuse).
      |
      | Gleichungen:
      |   Ω = 0
      |
      | Quelle: Hagl, R.: Elektrische Antriebstechnik. Hanser, München 2013
      mask Help:
      | Ruhendes Bezugssystem (Fundament, Gehäuse).
      | 
      | Gleichungen:
      |   Ω = 0
      | 
      | Quelle: Hagl, R.: Elektrische Antriebstechnik. Hanser, München 2013
      | 
      | Parameter und Wertebereiche:
      |   (keine)
      | 
      | Alle Standardwerte sind Beispielwerte (parameter/asm_standard.m), keine Datenblattwerte.
      | Spezifikation: doku/SPEC.md
      mask Display:
      | plot([0.05 0.95], [0.5 0.5]);
      | text(0.5, 0.5, 'Bezug', 'horizontalAlignment', 'center', 'verticalAlignment', 'middle', 'texmode', 'on');
      | port_label('LConn', 1, 'C', 'texmode', 'on');
  Reibung : Subsystem  Tag=asmlib:friction  mask(ASM-Bibliothek: Reibung){k_R=1e-3, M_C=0}
      mask prompts: k_R "Reibbeiwert k_R (viskos) [N·m·s/rad]"; M_C "Coulomb-Reibmoment M_C [N·m]"
      mask help:
      | Viskose und trockene Reibung (Lager, Lüfter des Motors).
      |
      | Gleichungen:
      |   M_R = k_R·Ω + M_C·sign(Ω)
      |
      | Quelle: Hagl, R.: Elektrische Antriebstechnik. Hanser, München 2013
      mask Help:
      | Viskose und trockene Reibung (Lager, Lüfter des Motors).
      | 
      | Gleichungen:
      |   M_R = k_R·Ω + M_C·sign(Ω)
      | 
      | Quelle: Hagl, R.: Elektrische Antriebstechnik. Hanser, München 2013
      | 
      | Parameter und Wertebereiche:
      |   k_R            ≥ 0  [N·m·s/rad]
      |   M_C            ≥ 0  [N·m]
      | 
      | Alle Standardwerte sind Beispielwerte (parameter/asm_standard.m), keine Datenblattwerte.
      | Spezifikation: doku/SPEC.md
      mask Display:
      | plot([0.05 0.95], [0.5 0.5]);
      | text(0.5, 0.5, 'k_R', 'horizontalAlignment', 'center', 'verticalAlignment', 'middle', 'texmode', 'on');
      | port_label('LConn', 1, 'R', 'texmode', 'on');
      | port_label('RConn', 1, 'C', 'texmode', 'on');
  Schwungmasse : Subsystem  Tag=asmlib:inertia  mask(ASM-Bibliothek: Schwungmasse){J=0.01, n0=0}
      mask prompts: J "Trägheitsmoment J [kg·m²]"; n0 "Anfangsdrehzahl n0 [1/min]"
      mask help:
      | Starre Schwungmasse (z. B. Trägheit der Arbeitsmaschine J_L).
      |
      | Gleichungen:
      |   J·dΩ/dt = Σ M
      |
      | Quelle: Hagl, R.: Elektrische Antriebstechnik. Hanser, München 2013; Densborn, Skript "DS-Asynchron-Motor" (DHBW Mannheim), Folie 68 (Hochlaufzeit)
      mask Help:
      | Starre Schwungmasse (z. B. Trägheit der Arbeitsmaschine J_L).
      | 
      | Gleichungen:
      |   J·dΩ/dt = Σ M
      | 
      | Quelle: Hagl, R.: Elektrische Antriebstechnik. Hanser, München 2013; Densborn, Skript "DS-Asynchron-Motor" (DHBW Mannheim), Folie 68 (Hochlaufzeit)
      | 
      | Parameter und Wertebereiche:
      |   J              > 0  [kg·m²]
      |   n0             endlich  [1/min]
      | 
      | Alle Standardwerte sind Beispielwerte (parameter/asm_standard.m), keine Datenblattwerte.
      | Spezifikation: doku/SPEC.md
      mask Display:
      | plot([0.05 0.95], [0.5 0.5]);
      | text(0.5, 0.5, 'J', 'horizontalAlignment', 'center', 'verticalAlignment', 'middle', 'texmode', 'on');
      | port_label('LConn', 1, 'R', 'texmode', 'on');
  Welle elastisch : Subsystem  Tag=asmlib:elastic_shaft  mask(ASM-Bibliothek: Welle elastisch){c_W=1e4, d_W=1}
      mask prompts: c_W "Drehsteifigkeit c [N·m/rad]"; d_W "Dämpfung d [N·m·s/rad]"
      mask help:
      | Drehelastische Welle bzw. Kupplung zwischen zwei Massen.
      |
      | Gleichungen:
      |   M = c·(ϑ_R − ϑ_C) + d·(Ω_R − Ω_C)
      |
      | Quelle: Hagl, R.: Elektrische Antriebstechnik. Hanser, München 2013
      mask Help:
      | Drehelastische Welle bzw. Kupplung zwischen zwei Massen.
      | 
      | Gleichungen:
      |   M = c·(ϑ_R − ϑ_C) + d·(Ω_R − Ω_C)
      | 
      | Quelle: Hagl, R.: Elektrische Antriebstechnik. Hanser, München 2013
      | 
      | Parameter und Wertebereiche:
      |   c_W            > 0  [N·m/rad]
      |   d_W            ≥ 0  [N·m·s/rad]
      | 
      | Alle Standardwerte sind Beispielwerte (parameter/asm_standard.m), keine Datenblattwerte.
      | Spezifikation: doku/SPEC.md
      mask Display:
      | plot([0.05 0.95], [0.5 0.5]);
      | text(0.5, 0.5, 'c, d', 'horizontalAlignment', 'center', 'verticalAlignment', 'middle', 'texmode', 'on');
      | port_label('LConn', 1, 'R', 'texmode', 'on');
      | port_label('RConn', 1, 'C', 'texmode', 'on');
